simulink model "airgear"  (R2024a)
settings: Solver=VariableStepAuto  StartTime=0.0  StopTime=2  RelTol=1e-3
values from neighbouring files (symbols this model uses):
  c = 1500    [air_gear.m]    (also in etude_influence_amortissement_c.m = c_list(i); etude_influence_raideur_k.m)
  F0 = 1000    [air_gear.m]
  k = 20000    [air_gear.m]    (also in etude_influence_amortissement_c.m; etude_influence_raideur_k.m = k_list(i))
  m = 100    [air_gear.m]    (also in etude_influence_amortissement_c.m; etude_influence_raideur_k.m)
settings Model: Creator=nnguy  LastModifiedBy=nnguy

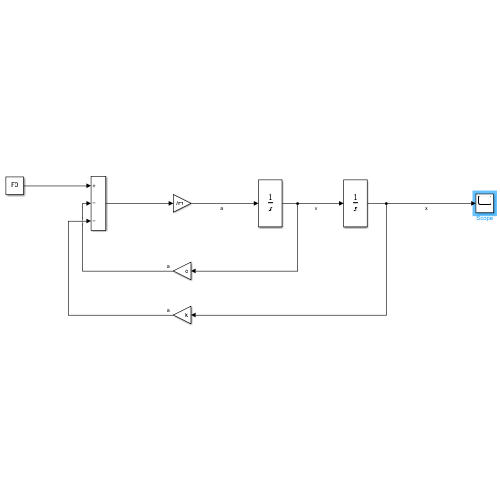
[thumbnail: Simulink's stored preview of the top-level diagram]
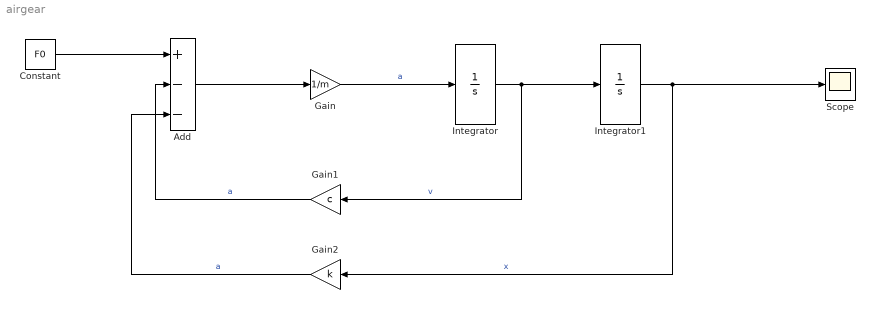
== system airgear ==
  Add : Sum  Inputs=+--
  Constant : Constant  Value=F0
  Gain : Gain  Gain=1/m
  Gain1 : Gain  Gain=c
  Gain2 : Gain  Gain=k
  Integrator : Integrator
  Integrator1 : Integrator
  Scope : Scope
  wires:
  Constant/1 -> Add/1
  Add/1 -> Gain/1
  Gain/1 -> Integrator/1  "a"
  Integrator/1 -> Gain1/1, Integrator1/1  "v"
  Gain1/1 -> Add/2  "a"
  Integrator1/1 -> Scope/1, Gain2/1  "x"
  Gain2/1 -> Add/3  "a"
